simulink model "PLL"  (R2026a)
settings: Solver=FixedStepDiscrete  StopTime=inf  FixedStep=Ts
model workspace (MATLAB code in the model file):
  | % Defaults for standalone use, from HPP_parameters. In HPP the Model
  | % block passes the instance's parameters as the argument "pll".
  | pDefault = HPP_parameters();
  | Ts = pDefault.sim.Ts;      % [s] simulation step
  | pll = pDefault.pll.asset;
  | clear pDefault
Description:
  | PLL, chosen per run (HPP_pll): MAF-PLL (1, SRF-PLL with moving-average prefilter) or Simple (2, the minimal SRF-PLL). Argument pll: see params/pllParameters.m.
settings Model: ParameterArgumentNames=pll  Creator=kjaer  LastModifiedBy=kjaer

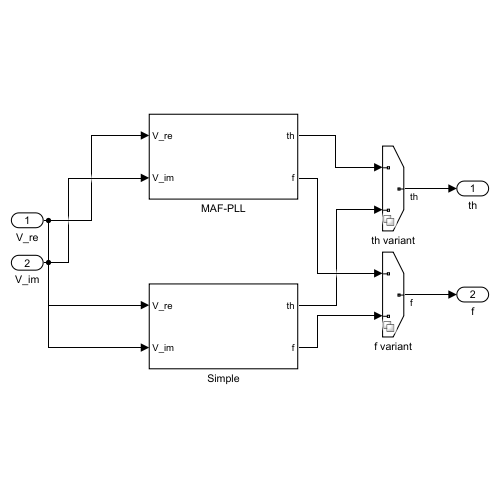
[thumbnail: Simulink's stored preview of the top-level diagram]
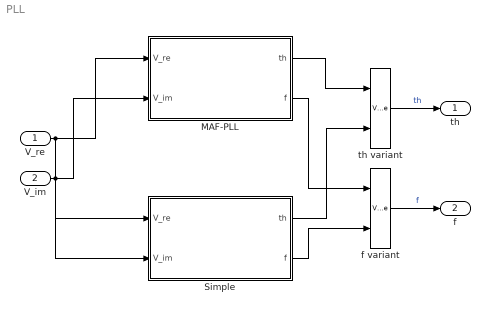
== system PLL ==
  V_re : Inport
  V_im : Inport  Port=2
  MAF-PLL : Subsystem  Description=SRF-PLL with moving-average prefilter (HPP_pll = 1)
  Simple : Subsystem  Description=the minimal SRF-PLL (HPP_pll = 2)
  f variant : VariantSource  VariantControls={HPP_pll == 1, HPP_pll == 2}
  th variant : VariantSource  VariantControls={HPP_pll == 1, HPP_pll == 2}
  th : Outport
  f : Outport  Port=2
  wires:
  V_re/1 -> MAF-PLL/1(V_re), Simple/1(V_re)
  V_im/1 -> MAF-PLL/2(V_im), Simple/2(V_im)
  MAF-PLL/1(th) -> th variant/1
  Simple/1(th) -> th variant/2
  MAF-PLL/2(f) -> f variant/1
  Simple/2(f) -> f variant/2
  th variant/1 -> th/1  "th"
  f variant/1 -> f/1  "f"

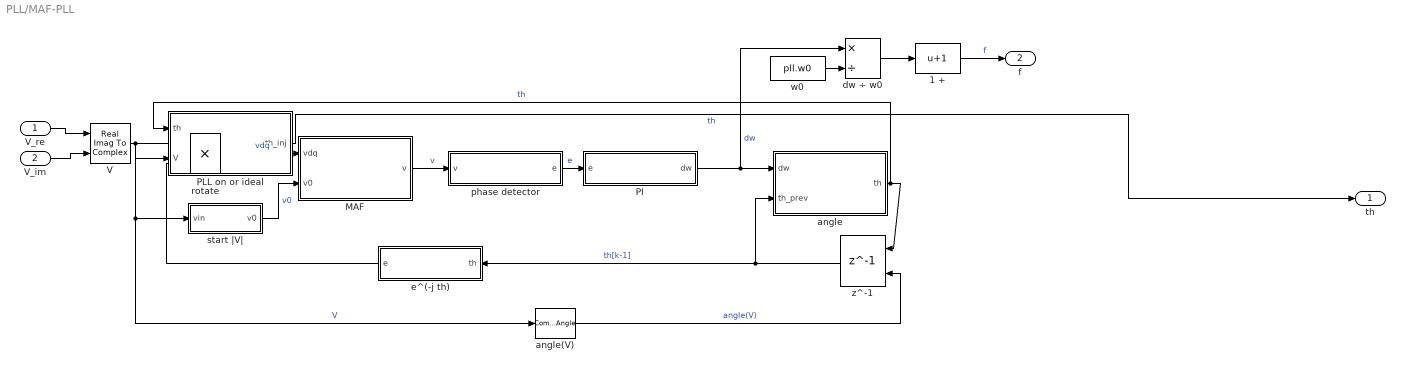
== system PLL/MAF-PLL ==
  V_re : Inport
  V_im : Inport  Port=2
  1 + : Bias  Bias=1  SaturateOnIntegerOverflow=off
  MAF : Subsystem  Description=Prefilter: moving average of the voltage in the PLL frame over Npre steps (MAF-PLL)
  PI : Subsystem  Description=dw = sat(kp e + xi), xi = sat(xi[k-1] + ki Ts e), +-5 Hz
  PLL on or ideal : Subsystem  Description=the angle the converter injects along: the PLL angle; on = 0 (ideal): the angle of V
  V : RealImagToComplex
  angle : Subsystem  Description=th = wrap(th[k-1] + Ts dw) to +-pi
  angle(V) : ComplexToMagnitudeAngle  Output=Angle
  dw ÷ w0 : Product  Inputs=*/
  e^(-j th) : Subsystem  Description=unit phasor of the angle, conjugated
  phase detector : Subsystem  Description=e = Im(v) / |v| = sin(angle error); 0 below 0.05 pu (held in a deep dip)
  rotate : Product
  start |V| : Subsystem  Description=start value of the prefilter: |V| (real)
  w0 : Constant  Value=pll.w0
  z^-1 : Delay  DelayLength=1  InitialConditionSource=Input port
      settings: InputPortMap=u0,p4
  th : Outport
  f : Outport  Port=2
  wires:
  1 +/1 -> f/1  "f"
  dw ÷ w0/1 -> 1 +/1
  w0/1 -> dw ÷ w0/2
  angle(V)/1 -> z^-1/2  "angle(V)"
  e^(-j th)/1(e) -> rotate/2
  z^-1/1 -> e^(-j th)/1(th), angle/2(th_prev)  "th[k-1]"
  angle/1(th) -> z^-1/1, PLL on or ideal/1(th)  "th"
  PI/1(dw) -> angle/1(dw), dw ÷ w0/1  "dw"
  phase detector/1(e) -> PI/1(e)  "e"
  MAF/1(v) -> phase detector/1(v)  "v"
  start |V|/1(v0) -> MAF/2(v0)  "v0"
  rotate/1 -> MAF/1(vdq)  "vdq"
  V/1 -> rotate/1, start |V|/1(vin), angle(V)/1, PLL on or ideal/2(V)  "V"
  V_im/1 -> V/2
  V_re/1 -> V/1
  PLL on or ideal/1(th_inj) -> th/1  "th"

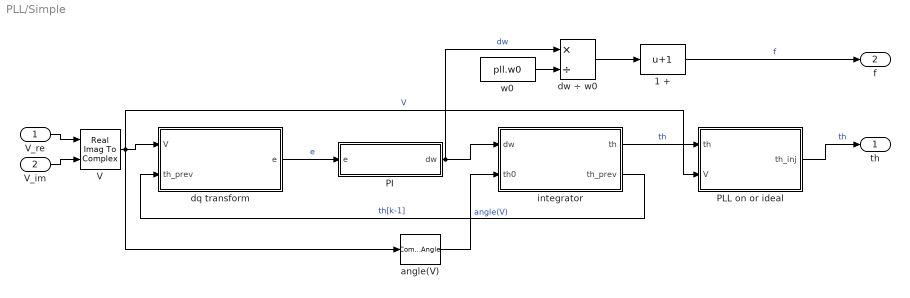
== system PLL/Simple ==
  V_re : Inport
  V_im : Inport  Port=2
  1 + : Bias  Bias=1  SaturateOnIntegerOverflow=off
  PI : Subsystem  Description=dw = kp e + xi, xi = xi[k-1] + ki Ts e (no limits)
  PLL on or ideal : Subsystem  Description=the angle the converter injects along: the PLL angle; on = 0 (ideal): the angle of V
  V : RealImagToComplex
  angle(V) : ComplexToMagnitudeAngle  Output=Angle
  dq transform : Subsystem  Description=vdq = V e^(-j th[k-1]); e = vq / max(|vdq|, 1e-3): the PI drives vq to zero
  dw ÷ w0 : Product  Inputs=*/
  integrator : Subsystem  Description=th = th[k-1] + Ts dw (not wrapped); th[k-1] starts at the angle of V
  w0 : Constant  Value=pll.w0
  th : Outport
  f : Outport  Port=2
  wires:
  V_re/1 -> V/1
  V_im/1 -> V/2
  V/1 -> dq transform/1(V), PLL on or ideal/2(V), angle(V)/1  "V"
  dq transform/1(e) -> PI/1(e)  "e"
  PI/1(dw) -> integrator/1(dw), dw ÷ w0/1  "dw"
  integrator/1(th) -> PLL on or ideal/1(th)  "th"
  PLL on or ideal/1(th_inj) -> th/1  "th"
  integrator/2(th_prev) -> dq transform/2(th_prev)  "th[k-1]"
  angle(V)/1 -> integrator/2(th0)  "angle(V)"
  w0/1 -> dw ÷ w0/2
  dw ÷ w0/1 -> 1 +/1
  1 +/1 -> f/1  "f"

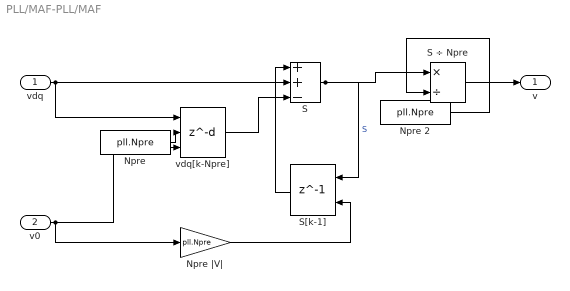
== system PLL/MAF-PLL/MAF ==
  vdq : Inport
  v0 : Inport  Port=2
  Npre : Constant  Value=pll.Npre
  Npre 2 : Constant  Value=pll.Npre
  Npre |V| : Gain  Gain=pll.Npre
  S : Sum  Inputs=++-
  S ÷ Npre : Product  Inputs=*/
  S[k-1] : Delay  DelayLength=1  InitialConditionSource=Input port
      settings: InputPortMap=u0,p4
  vdq[k-Npre] : Delay  DelayLengthSource=Input port  DelayLengthUpperLimit=50  InitialConditionSource=Input port
      settings: InputPortMap=u0,p1,p4
  v : Outport
  wires:
  vdq/1 -> S/2, vdq[k-Npre]/1
  Npre/1 -> vdq[k-Npre]/2
  v0/1 -> vdq[k-Npre]/3, Npre |V|/1
  vdq[k-Npre]/1 -> S/3
  S/1 -> S ÷ Npre/1, S[k-1]/1  "S"
  Npre 2/1 -> S ÷ Npre/2
  S ÷ Npre/1 -> v/1
  S[k-1]/1 -> S/1
  Npre |V|/1 -> S[k-1]/2

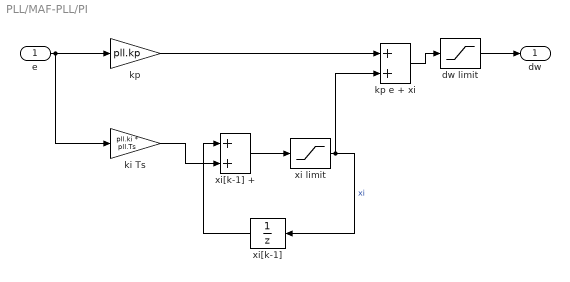
== system PLL/MAF-PLL/PI ==
  e : Inport
  dw limit : Saturate  UpperLimit=pll.wlim  LowerLimit=-pll.wlim
  ki Ts : Gain  Gain=pll.ki * pll.Ts
  kp : Gain  Gain=pll.kp
  kp e + xi : Sum
  xi limit : Saturate  UpperLimit=pll.wlim  LowerLimit=-pll.wlim
  xi[k-1] : UnitDelay  SampleTime=-1
  xi[k-1] + : Sum
  dw : Outport
  wires:
  e/1 -> kp/1, ki Ts/1
  ki Ts/1 -> xi[k-1] +/2
  xi[k-1] +/1 -> xi limit/1
  xi limit/1 -> xi[k-1]/1, kp e + xi/2  "xi"
  xi[k-1]/1 -> xi[k-1] +/1
  kp/1 -> kp e + xi/1
  kp e + xi/1 -> dw limit/1
  dw limit/1 -> dw/1

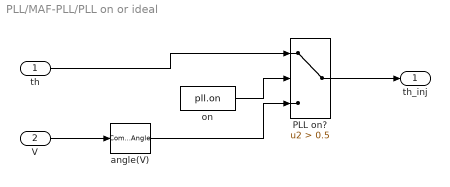
== system PLL/MAF-PLL/PLL on or ideal ==
  th : Inport
  V : Inport  Port=2
  PLL on? : Switch  Criteria=u2 > Threshold  Threshold=0.5  SaturateOnIntegerOverflow=off  InputSameDT=off
  angle(V) : ComplexToMagnitudeAngle  Output=Angle
  on : Constant  Value=pll.on
  th_inj : Outport
  wires:
  th/1 -> PLL on?/1
  on/1 -> PLL on?/2
  V/1 -> angle(V)/1
  angle(V)/1 -> PLL on?/3
  PLL on?/1 -> th_inj/1

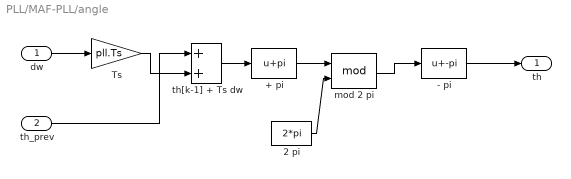
== system PLL/MAF-PLL/angle ==
  dw : Inport
  th_prev : Inport  Port=2
  + pi : Bias  Bias=pi  SaturateOnIntegerOverflow=off
  - pi : Bias  Bias=-pi  SaturateOnIntegerOverflow=off
  2 pi : Constant  Value=2*pi
  Ts : Gain  Gain=pll.Ts
  mod 2 pi : Math  Operator=mod
  th[k-1] + Ts dw : Sum
  th : Outport
  wires:
  dw/1 -> Ts/1
  th_prev/1 -> th[k-1] + Ts dw/1
  Ts/1 -> th[k-1] + Ts dw/2
  th[k-1] + Ts dw/1 -> + pi/1
  + pi/1 -> mod 2 pi/1
  2 pi/1 -> mod 2 pi/2
  mod 2 pi/1 -> - pi/1
  - pi/1 -> th/1

== system PLL/MAF-PLL/e^(-j th) ==
  th : Inport
  conj : Math  Operator=conj
  e^(j th) : MagnitudeAngleToComplex  Input=Angle  ConstantPart=1
  e : Outport
  wires:
  th/1 -> e^(j th)/1
  e^(j th)/1 -> conj/1
  conj/1 -> e/1

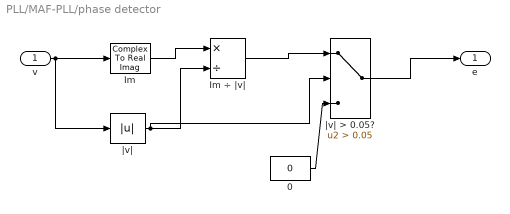
== system PLL/MAF-PLL/phase detector ==
  v : Inport
  0 : Constant  Value=0
  Im : ComplexToRealImag  Output=Imag
  Im ÷ |v| : Product  Inputs=*/
  |v| : Abs  SaturateOnIntegerOverflow=off
  |v| > 0.05? : Switch  Criteria=u2 > Threshold  Threshold=0.05  SaturateOnIntegerOverflow=off  InputSameDT=off
  e : Outport
  wires:
  v/1 -> Im/1, |v|/1
  Im/1 -> Im ÷ |v|/1
  |v|/1 -> Im ÷ |v|/2, |v| > 0.05?/2
  Im ÷ |v|/1 -> |v| > 0.05?/1
  0/1 -> |v| > 0.05?/3
  |v| > 0.05?/1 -> e/1

== system PLL/MAF-PLL/start |V| ==
  vin : Inport
  0 : Constant  Value=0
  |V| : Abs  SaturateOnIntegerOverflow=off
  |V| + j0 : RealImagToComplex
  v0 : Outport
  wires:
  vin/1 -> |V|/1
  |V|/1 -> |V| + j0/1
  0/1 -> |V| + j0/2
  |V| + j0/1 -> v0/1

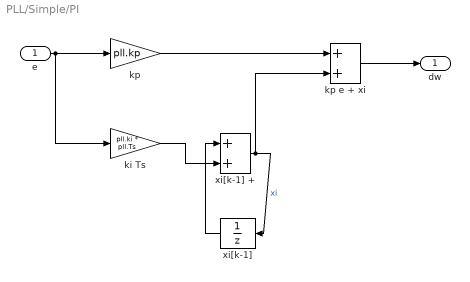
== system PLL/Simple/PI ==
  e : Inport
  ki Ts : Gain  Gain=pll.ki * pll.Ts
  kp : Gain  Gain=pll.kp
  kp e + xi : Sum
  xi[k-1] : UnitDelay  SampleTime=-1
  xi[k-1] + : Sum
  dw : Outport
  wires:
  e/1 -> kp/1, ki Ts/1
  ki Ts/1 -> xi[k-1] +/2
  xi[k-1] +/1 -> xi[k-1]/1, kp e + xi/2  "xi"
  xi[k-1]/1 -> xi[k-1] +/1
  kp/1 -> kp e + xi/1
  kp e + xi/1 -> dw/1

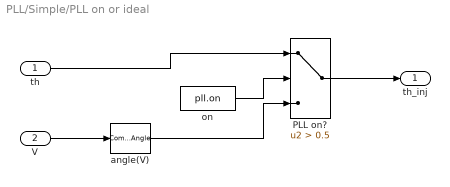
== system PLL/Simple/PLL on or ideal ==
  th : Inport
  V : Inport  Port=2
  PLL on? : Switch  Criteria=u2 > Threshold  Threshold=0.5  SaturateOnIntegerOverflow=off  InputSameDT=off
  angle(V) : ComplexToMagnitudeAngle  Output=Angle
  on : Constant  Value=pll.on
  th_inj : Outport
  wires:
  th/1 -> PLL on?/1
  on/1 -> PLL on?/2
  V/1 -> angle(V)/1
  angle(V)/1 -> PLL on?/3
  PLL on?/1 -> th_inj/1

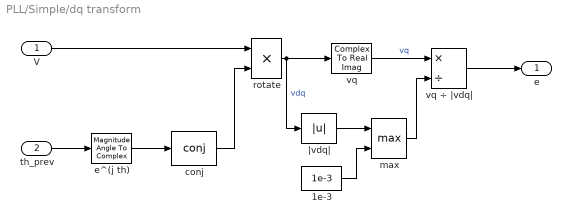
== system PLL/Simple/dq transform ==
  V : Inport
  th_prev : Inport  Port=2
  1e-3 : Constant  Value=1e-3
  conj : Math  Operator=conj
  e^(j th) : MagnitudeAngleToComplex  Input=Angle  ConstantPart=1
  max : MinMax  Function=max  Inputs=2
  rotate : Product
  vq : ComplexToRealImag  Output=Imag
  vq ÷ |vdq| : Product  Inputs=*/
  |vdq| : Abs  SaturateOnIntegerOverflow=off
  e : Outport
  wires:
  th_prev/1 -> e^(j th)/1
  e^(j th)/1 -> conj/1
  V/1 -> rotate/1
  conj/1 -> rotate/2
  rotate/1 -> vq/1, |vdq|/1  "vdq"
  |vdq|/1 -> max/1
  1e-3/1 -> max/2
  vq/1 -> vq ÷ |vdq|/1  "vq"
  max/1 -> vq ÷ |vdq|/2
  vq ÷ |vdq|/1 -> e/1

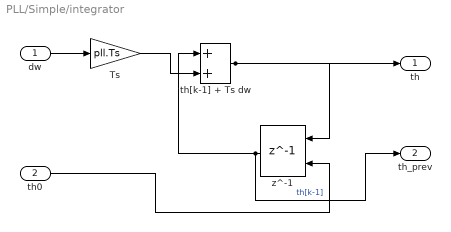
== system PLL/Simple/integrator ==
  dw : Inport
  th0 : Inport  Port=2
  Ts : Gain  Gain=pll.Ts
  th[k-1] + Ts dw : Sum
  z^-1 : Delay  DelayLength=1  InitialConditionSource=Input port
      settings: InputPortMap=u0,p4
  th : Outport
  th_prev : Outport  Port=2
  wires:
  dw/1 -> Ts/1
  Ts/1 -> th[k-1] + Ts dw/2
  th[k-1] + Ts dw/1 -> th/1, z^-1/1
  th0/1 -> z^-1/2
  z^-1/1 -> th[k-1] + Ts dw/1, th_prev/1  "th[k-1]"
